simulink model "model_simulink_lab1_1"  (R2026a)
settings: Solver=VariableStepAuto  StopTime=10
undefined symbols (not defined in the file or in its folder): Blocking, Non
libraries: amg_usbconverter_n_connect_lib x2
settings Model: Creator=rosva  LastModifiedBy=rosva

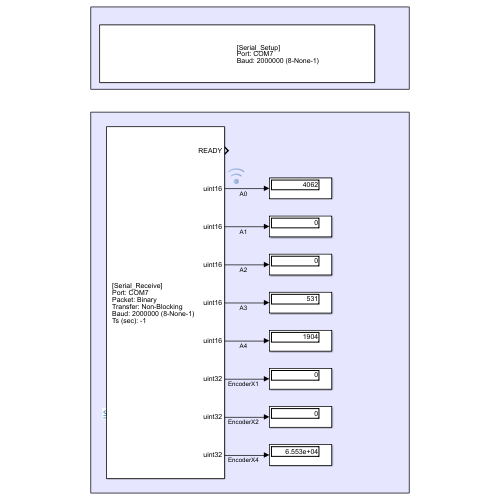
[thumbnail: Simulink's stored preview of the top-level diagram]
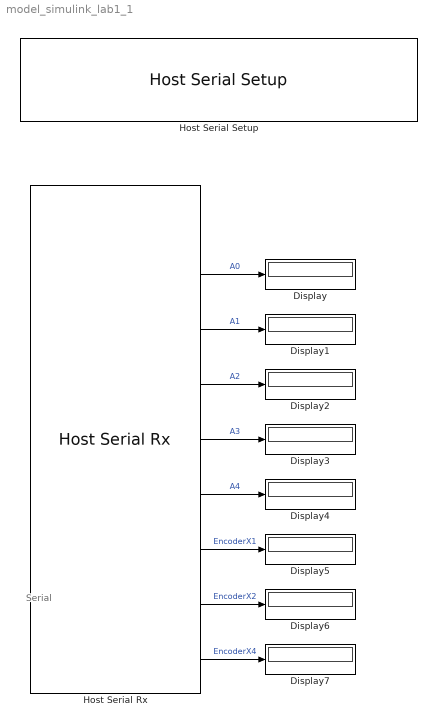
== system model_simulink_lab1_1 ==
  note: Serial
  Display{,1..7} (8 alike) : Display
  Host Serial Rx : amg_usbconverter_n_connect_lib/Host Serial Rx  conf=rx  port=COM7  baudrate=2000000  databits=8  parity=None  stopbit=1  flowcontrol=None  transfer=Non-Blocking  timeout=5  packetmode=Binary  enableinitialvalues=off  initialvalues=[]  binheader='25'  binterminator='4E 4E'  porttype_double=0  porttype_single=0  porttype_int8=0  porttype_uint8=0  porttype_int16=0  porttype_uint16=5  porttype_int32=0  porttype_uint32=3  asciiformat='%d,%f'  rx_asciiterminator="CRLF (0x0D 0x0A - \"\\r\\n\")"  tx_asciiterminator="CRLF (0x0D 0x0A - \"\\r\\n\")"  sampletime=0.001  enablecustomportlabel=off  cinputportlabel=0  coutputportlabel=A  portpinstr=0  blockid=HostSerialRx  inputporttype=[]  inputportwidth=[]  inputportlabel={}  outputporttype=[3 5 5 5 5 5 7 7 7]  outputportwidth=[1 1 1 1 1 1 1 1 1]  outputportlabel={'READY','uint16','uint16','uint16','uint16','uint16','uint32','uint32','uint32'}  compat=0  optionstring=[]  autoport='COM7'
  Host Serial Setup : amg_usbconverter_n_connect_lib/Host Serial Setup  conf=setup  port=COM7  baudrate=2000000  databits=8  parity=None  stopbit=1  flowcontrol=None  transfer=Blocking  timeout=2  packetmode=Binary  initialvalues=[]  binheader='7E 7E'  binterminator='03 03'  porttype_double=0  porttype_single=1  porttype_int8=0  porttype_uint8=0  porttype_int16=0  porttype_uint16=0  porttype_int32=0  porttype_uint32=2  asciiformat='%d %u %x'  rx_asciiterminator="CRLF (0x0D 0x0A - \"\\r\\n\")"  tx_asciiterminator="CRLF (0x0D 0x0A - \"\\r\\n\")"  sampletime=-1  enablecustomportlabel=off  cinputportlabel=0  coutputportlabel=A  portpinstr=0  blockid=HostSerialSetup  inputporttype=[]  inputportwidth=[]  inputportlabel={}  outputporttype=[]  outputportwidth=[]  outputportlabel={}  compat=0  optionstring=[]  autoport='COM7'
  wires:
  Host Serial Rx/5 -> Display3/1  "A3"
  Host Serial Rx/7 -> Display5/1  "EncoderX1"
  Host Serial Rx/4 -> Display2/1  "A2"
  Host Serial Rx/3 -> Display1/1  "A1"
  Host Serial Rx/6 -> Display4/1  "A4"
  Host Serial Rx/9 -> Display7/1  "EncoderX4"
  Host Serial Rx/2 -> Display/1  "A0"
  Host Serial Rx/8 -> Display6/1  "EncoderX2"
